simulink model "EV_BMS_Simscape"  (R2026b)
settings: Solver=ode23t  StopTime=5000  MaxStep=1
values from neighbouring files (symbols this model uses):
  thr = struct('pack', Inf, 'curr', Inf, 'innov', Inf, 'noise', Inf)    [simulate_charging_simulink.m]
undefined symbols (not defined in the file or in its folder): ac, bp, defence, seed_atk, seed_meas, seed_u
libraries: nesl_utility x18, evbms_lib x5, fl_lib x1
settings Model: Creator=yugagarwal105  LastModifiedBy=yugagarwal105
settings SimscapeCC: SimscapeLogType=all  SimscapeNominalValues="[{\"value\":\"1\",\"unit\":\"A\"},{\"value\":\"1\",\"unit\":\"bar\"},{\"value\":\"1\",\"unit\":\"cm^2\"},{\"value\":\"1\",\"unit\":\"cm^3/s\"},{\"value\":\"1\",\"unit\":\"kJ/kg\"},{\"value\":\"1\",\"unit\":\"kW\"},{\"value\":\"1\",\"unit\":\"l\"},{\"value\":\"1\",\"unit\":\"N\"},{\"value\":\"1\",\"unit\":\"N*m\"},{\"value\":\"1\",\"unit\":\"V\"},{\"value\":\"0.001\",\"unit\":\"Wb\"}]"  SimscapeUseEnergyAccounting=off

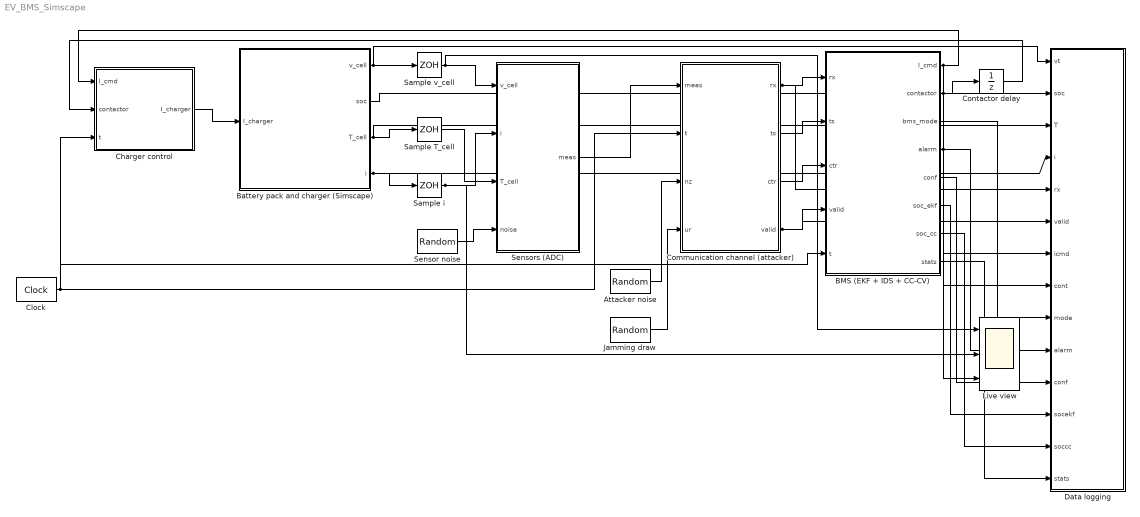
== system EV_BMS_Simscape ==
  Attacker noise : RandomNumber  Mean=zeros(1,4)  Variance=ones(1,4)  Seed=seed_atk  SampleTime=1
  BMS (EKF + IDS + CC-CV) : MATLAB Function  TreatAsAtomicUnit=on
  Battery pack and charger (Simscape) : Subsystem
      mask Display: port_label('input',1,'I charger');port_label('output',1,'V cells');port_label('output',2,'SoC');port_label('output',3,'T cells');port_label('output',4,'I pack');
  Charger control : Subsystem
      mask Display: port_label('input',1,'I cmd');port_label('input',2,'contactor');port_label('input',3,'t');port_label('output',1,'I');
  Clock : DigitalClock
  Communication channel (attacker) : MATLAB Function  TreatAsAtomicUnit=on
  Contactor delay : UnitDelay  InitialCondition=1
  Data logging : Subsystem
      mask Display: disp('Data logging\n(To Workspace)');
  Jamming draw : UniformRandomNumber  Minimum=0  Seed=seed_u  SampleTime=1
  Live view : Scope  NumInputPorts=3
  Sample T_cell : ZeroOrderHold
  Sample i : ZeroOrderHold
  Sample v_cell : ZeroOrderHold
  Sensor noise : RandomNumber  Mean=zeros(1,10)  Variance=ones(1,10)  Seed=seed_meas  SampleTime=1
  Sensors (ADC) : MATLAB Function  TreatAsAtomicUnit=on
  wires:
  Charger control/1(I_charger) -> Battery pack and charger (Simscape)/1(I_charger)
  Battery pack and charger (Simscape)/1(v_cell) -> Sample v_cell/1, Data logging/1(vt)
  Battery pack and charger (Simscape)/4(i) -> Sample i/1, Data logging/4(i)
  Battery pack and charger (Simscape)/3(T_cell) -> Sample T_cell/1, Data logging/3(T)
  Sample v_cell/1 -> Sensors (ADC)/1(v_cell), Live view/1
  Sample i/1 -> Sensors (ADC)/2(i), Live view/2
  Sample T_cell/1 -> Sensors (ADC)/3(T_cell)
  Sensor noise/1 -> Sensors (ADC)/4(noise)
  Sensors (ADC)/1(meas) -> Communication channel (attacker)/1(meas)
  Clock/1 -> Communication channel (attacker)/2(t), BMS (EKF + IDS + CC-CV)/5(t), Charger control/3(t)
  Attacker noise/1 -> Communication channel (attacker)/3(nz)
  Jamming draw/1 -> Communication channel (attacker)/4(ur)
  Communication channel (attacker)/1(rx) -> BMS (EKF + IDS + CC-CV)/1(rx), Data logging/5(rx)
  Communication channel (attacker)/2(ts) -> BMS (EKF + IDS + CC-CV)/2(ts)
  Communication channel (attacker)/3(ctr) -> BMS (EKF + IDS + CC-CV)/3(ctr)
  Communication channel (attacker)/4(valid) -> BMS (EKF + IDS + CC-CV)/4(valid), Data logging/6(valid)
  BMS (EKF + IDS + CC-CV)/1(I_cmd) -> Charger control/1(I_cmd), Data logging/7(icmd)
  BMS (EKF + IDS + CC-CV)/2(contactor) -> Contactor delay/1, Data logging/8(cont)
  Contactor delay/1 -> Charger control/2(contactor)
  Battery pack and charger (Simscape)/2(soc) -> Data logging/2(soc)
  BMS (EKF + IDS + CC-CV)/3(bms_mode) -> Data logging/9(mode)
  BMS (EKF + IDS + CC-CV)/4(alarm) -> Data logging/10(alarm), Live view/3
  BMS (EKF + IDS + CC-CV)/5(conf) -> Data logging/11(conf)
  BMS (EKF + IDS + CC-CV)/6(soc_ekf) -> Data logging/12(socekf)
  BMS (EKF + IDS + CC-CV)/7(soc_cc) -> Data logging/13(soccc)
  BMS (EKF + IDS + CC-CV)/8(stats) -> Data logging/14(stats)

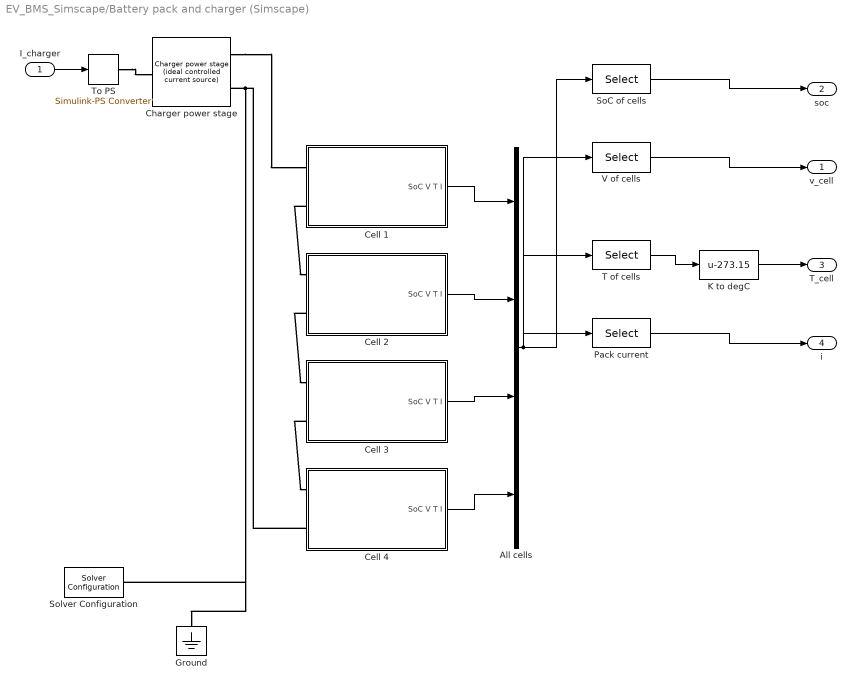
== system EV_BMS_Simscape/Battery pack and charger (Simscape) ==
  I_charger : Inport
  All cells : Mux
  Cell 1 : Subsystem
      mask Display: disp('Li-ion cell 1\nSoC0 = 0.20');port_label('LConn',1,'+');port_label('LConn',2,'-');
  Cell 2 : Subsystem
      mask Display: disp('Li-ion cell 2\nSoC0 = 0.24');port_label('LConn',1,'+');port_label('LConn',2,'-');
  Cell 3 : Subsystem
      mask Display: disp('Li-ion cell 3\nSoC0 = 0.21');port_label('LConn',1,'+');port_label('LConn',2,'-');
  Cell 4 : Subsystem
      mask Display: disp('Li-ion cell 4\nSoC0 = 0.20');port_label('LConn',1,'+');port_label('LConn',2,'-');
  Charger power stage : evbms_lib/Charger power stage (ideal controlled current source)  i_specify=off  i_priority=None  i=0 A  i_nominal_specify=off  i_nominal_value=1  i_nominal_unit=A  v_specify=off  v_priority=None  v=0 V  v_nominal_specify=off  v_nominal_value=1  v_nominal_unit=V
  Ground : fl_lib/Electrical/Electrical Elements/Electrical Reference
  K to degC : Bias  Bias=-273.15  SaturateOnIntegerOverflow=off
  Pack current : Selector  InputPortWidth=16  IndexOptions=Index vector (dialog)  Indices=[4]  OutputSizes=1
  SoC of cells : Selector  InputPortWidth=16  IndexOptions=Index vector (dialog)  Indices=[1 5 9 13]  OutputSizes=1
  Solver Configuration : nesl_utility/Solver Configuration  PhysicalDomain=network_engine_domain  SubClassName=solver  LeftPortType=input  RightPortType=generic  Tones=[]  Harmonics=[]  SimulateNoise=off  Profile=off  UseLocalSampling=off  EnableSwitchedLinearOptims=on  FrequencyDomain=off  UseCCode=off  RelTol=0.001  AbsTol=0.001  MinStep=1e-09  ToWorkspace=off  RevertToSquareIcSolve=off  NumHomotopyIterations=100  PhasorMode=off  PhasorModeNumHarmonics=1  ConsistencySolver=NEWTON_XTOL_AFTER_FTOL  CanonicalOrdering=CANONICAL  OptimizeIntermediates=OPTIMIZED  MulticoreSolverChoice=BACKWARD_EULER  IndexReductionMethod=DerivativeReplacement  DoDC=off  ResidualTolerance=1e-09  ConsistencyTolSource=GLOBAL  ConsistencyAbsTol=0.001  ConsistencyRelTol=0.001  ConsistencyTolFactor=0.001  UseLocalSolver=off  LocalSolverChoice=NE_BACKWARD_EULER_ADVANCER  ResolveIndetEquations=on  FunctionEvalNumThread=1  LocalSolverSampleTime=0.001  DoFixedCost=off  MaxNonlinIter=3  MaxModeIter=2  ComputeImpulses=off  ImpulseIterations=2  LinearAlgebra=auto  LinearAlgebraNumThread=0  EquationFormulation=NE_TIME_EF  DelaysMemoryBudget=1024  AutomaticFiltering=on  FilteringTimeConstant=0.001  PartitionStorageMethod=AS_NEEDED  PartitionMemoryBudget=1024  PartitionMethod=BALANCED  MultibodyUseLocalSolver=off  MultibodyLocalSolverChoice=ODE1  MultibodyLocalSolverSampleTime=0.001
  T of cells : Selector  InputPortWidth=16  IndexOptions=Index vector (dialog)  Indices=[3 7 11 15]  OutputSizes=1
  To PS : nesl_utility/Simulink-PS Converter  PhysicalDomain=network_engine_domain  SubClassName=ps_input  LeftPortType=input  RightPortType=output  PseudoPeriodic=off  Frequencies=[]  NoiseDistribution=none  NoiseParameters=[]  Unit=A  AffineConversion=off  FilteringAndDerivatives=provide  SimscapeFilterOrder=1  InputFilterTimeConstant=0.001  UdotUserProvided=0
  V of cells : Selector  InputPortWidth=16  IndexOptions=Index vector (dialog)  Indices=[2 6 10 14]  OutputSizes=1
  v_cell : Outport
  soc : Outport  Port=2
  T_cell : Outport  Port=3
  i : Outport  Port=4
  wires:
  I_charger/1 -> To PS/1
  Cell 1/1(SoC V T I) -> All cells/1
  Cell 2/1(SoC V T I) -> All cells/2
  Cell 3/1(SoC V T I) -> All cells/3
  Cell 4/1(SoC V T I) -> All cells/4
  All cells/1 -> SoC of cells/1, V of cells/1, T of cells/1, Pack current/1
  SoC of cells/1 -> soc/1
  V of cells/1 -> v_cell/1
  T of cells/1 -> K to degC/1
  K to degC/1 -> T_cell/1
  Pack current/1 -> i/1
  connections:
  To PS/RConn1 -- Charger power stage/LConn1
  Charger power stage/RConn1 -- Cell 1/LConn1
  Cell 1/LConn2 -- Cell 2/LConn1
  Cell 2/LConn2 -- Cell 3/LConn1
  Cell 3/LConn2 -- Cell 4/LConn1
  Cell 4/LConn2 -- Ground/LConn1 -- Charger power stage/RConn2 -- Solver Configuration/RConn1

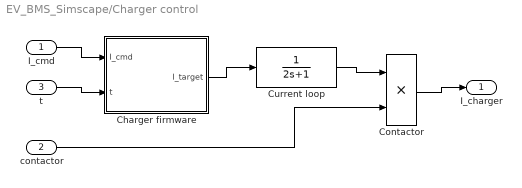
== system EV_BMS_Simscape/Charger control ==
  I_cmd : Inport
  contactor : Inport  Port=2
  t : Inport  Port=3
  Charger firmware : MATLAB Function  TreatAsAtomicUnit=on
  Contactor : Product
  Current loop : TransferFcn  Numerator=1  Denominator=[2 1]
  I_charger : Outport
  wires:
  I_cmd/1 -> Charger firmware/1(I_cmd)
  t/1 -> Charger firmware/2(t)
  Charger firmware/1(I_target) -> Current loop/1
  Current loop/1 -> Contactor/1
  contactor/1 -> Contactor/2
  Contactor/1 -> I_charger/1

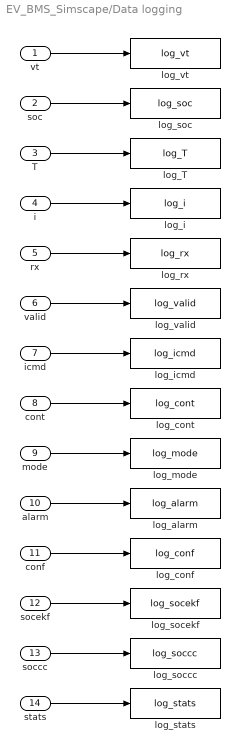
== system EV_BMS_Simscape/Data logging ==
  vt : Inport
  soc : Inport  Port=2
  T : Inport  Port=3
  i : Inport  Port=4
  rx : Inport  Port=5
  valid : Inport  Port=6
  icmd : Inport  Port=7
  cont : Inport  Port=8
  mode : Inport  Port=9
  alarm : Inport  Port=10
  conf : Inport  Port=11
  socekf : Inport  Port=12
  soccc : Inport  Port=13
  stats : Inport  Port=14
  log_T : ToWorkspace  VariableName=log_T  SampleTime=1
      settings: Save2DSignal=2-D array (concatenate along first dimension)
  log_alarm : ToWorkspace  VariableName=log_alarm  SampleTime=1
      settings: Save2DSignal=2-D array (concatenate along first dimension)
  log_conf : ToWorkspace  VariableName=log_conf  SampleTime=1
      settings: Save2DSignal=2-D array (concatenate along first dimension)
  log_cont : ToWorkspace  VariableName=log_cont  SampleTime=1
      settings: Save2DSignal=2-D array (concatenate along first dimension)
  log_i : ToWorkspace  VariableName=log_i  SampleTime=1
      settings: Save2DSignal=2-D array (concatenate along first dimension)
  log_icmd : ToWorkspace  VariableName=log_icmd  SampleTime=1
      settings: Save2DSignal=2-D array (concatenate along first dimension)
  log_mode : ToWorkspace  VariableName=log_mode  SampleTime=1
      settings: Save2DSignal=2-D array (concatenate along first dimension)
  log_rx : ToWorkspace  VariableName=log_rx  SampleTime=1
      settings: Save2DSignal=2-D array (concatenate along first dimension)
  log_soc : ToWorkspace  VariableName=log_soc  SampleTime=1
      settings: Save2DSignal=2-D array (concatenate along first dimension)
  log_soccc : ToWorkspace  VariableName=log_soccc  SampleTime=1
      settings: Save2DSignal=2-D array (concatenate along first dimension)
  log_socekf : ToWorkspace  VariableName=log_socekf  SampleTime=1
      settings: Save2DSignal=2-D array (concatenate along first dimension)
  log_stats : ToWorkspace  VariableName=log_stats  SampleTime=1
      settings: Save2DSignal=2-D array (concatenate along first dimension)
  log_valid : ToWorkspace  VariableName=log_valid  SampleTime=1
      settings: Save2DSignal=2-D array (concatenate along first dimension)
  log_vt : ToWorkspace  VariableName=log_vt  SampleTime=1
      settings: Save2DSignal=2-D array (concatenate along first dimension)
  wires:
  vt/1 -> log_vt/1
  soc/1 -> log_soc/1
  T/1 -> log_T/1
  i/1 -> log_i/1
  rx/1 -> log_rx/1
  valid/1 -> log_valid/1
  icmd/1 -> log_icmd/1
  cont/1 -> log_cont/1
  mode/1 -> log_mode/1
  alarm/1 -> log_alarm/1
  conf/1 -> log_conf/1
  socekf/1 -> log_socekf/1
  soccc/1 -> log_soccc/1
  stats/1 -> log_stats/1

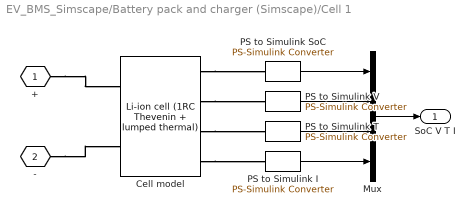
== system EV_BMS_Simscape/Battery pack and charger (Simscape)/Cell 1 ==
  Cell model : evbms_lib/Li-ion cell (1RC Thevenin + lumped thermal)  Q=2.6 A*hr  R0=0.03 Ohm  R1=0.015 Ohm  C1=2000 F  soc0=0.2  soc_bp=[-.1, 0, .05, .1, .2, .3, .4, .5, .6, .7, .8, .9, .95, 1, 1.5]  ocv_tab=[2.8, 3, 3.35, 3.45, 3.55, 3.62, 3.68, 3.74, 3.82, 3.9, 3.98, 4.07, 4.12, 4.2, 5.2] V  Cth=40 J/K  hA=0.05 W/K  Tamb=298.15 K  k_oc=5 W/A  i_specify=off  i_priority=None  i=0 A  i_nominal_specify=off  i_nominal_value=1  i_nominal_unit=A  v_specify=off  v_priority=None  v=0 V  v_nominal_specify=off  v_nominal_value=1  v_nominal_unit=V  v1_specify=off  v1_priority=High  v1=0 V  v1_nominal_specify=off  v1_nominal_value=1  v1_nominal_unit=V  dz_specify=off  dz_priority=High  dz=0  dz_nominal_specify=off  dz_nominal_value=1  dz_nominal_unit=1  dT_specify=off  dT_priority=High  dT=0 K  dT_nominal_specify=off  dT_nominal_value=1  dT_nominal_unit=K
  Mux : Mux
  PS to Simulink I : nesl_utility/PS-Simulink Converter  PhysicalDomain=network_engine_domain  SubClassName=ps_output  LeftPortType=input  RightPortType=output  PseudoPeriodic=off  Frequencies=[]  VectorFormat=inherit  Unit=A  AffineConversion=off
  PS to Simulink SoC : nesl_utility/PS-Simulink Converter  PhysicalDomain=network_engine_domain  SubClassName=ps_output  LeftPortType=input  RightPortType=output  PseudoPeriodic=off  Frequencies=[]  VectorFormat=inherit  Unit=1  AffineConversion=off
  PS to Simulink T : nesl_utility/PS-Simulink Converter  PhysicalDomain=network_engine_domain  SubClassName=ps_output  LeftPortType=input  RightPortType=output  PseudoPeriodic=off  Frequencies=[]  VectorFormat=inherit  Unit=K  AffineConversion=off
  PS to Simulink V : nesl_utility/PS-Simulink Converter  PhysicalDomain=network_engine_domain  SubClassName=ps_output  LeftPortType=input  RightPortType=output  PseudoPeriodic=off  Frequencies=[]  VectorFormat=inherit  Unit=V  AffineConversion=off
  + : PMIOPort  Side=Left
  - : PMIOPort  Port=2  Side=Left
  SoC V T I : Outport
  wires:
  PS to Simulink SoC/1 -> Mux/1
  PS to Simulink V/1 -> Mux/2
  PS to Simulink T/1 -> Mux/3
  PS to Simulink I/1 -> Mux/4
  Mux/1 -> SoC V T I/1
  connections:
  +/RConn1 -- Cell model/LConn1
  -/RConn1 -- Cell model/LConn2
  Cell model/RConn1 -- PS to Simulink SoC/LConn1
  Cell model/RConn2 -- PS to Simulink V/LConn1
  Cell model/RConn3 -- PS to Simulink T/LConn1
  Cell model/RConn4 -- PS to Simulink I/LConn1

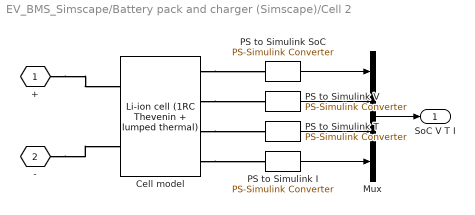
== system EV_BMS_Simscape/Battery pack and charger (Simscape)/Cell 2 ==
  Cell model : evbms_lib/Li-ion cell (1RC Thevenin + lumped thermal)  Q=2.548 A*hr  R0=0.0315 Ohm  R1=0.0156 Ohm  C1=1940 F  soc0=0.24  soc_bp=[-.1, 0, .05, .1, .2, .3, .4, .5, .6, .7, .8, .9, .95, 1, 1.5]  ocv_tab=[2.8, 3, 3.35, 3.45, 3.55, 3.62, 3.68, 3.74, 3.82, 3.9, 3.98, 4.07, 4.12, 4.2, 5.2] V  Cth=40 J/K  hA=0.05 W/K  Tamb=298.15 K  k_oc=5 W/A  i_specify=off  i_priority=None  i=0 A  i_nominal_specify=off  i_nominal_value=1  i_nominal_unit=A  v_specify=off  v_priority=None  v=0 V  v_nominal_specify=off  v_nominal_value=1  v_nominal_unit=V  v1_specify=off  v1_priority=High  v1=0 V  v1_nominal_specify=off  v1_nominal_value=1  v1_nominal_unit=V  dz_specify=off  dz_priority=High  dz=0  dz_nominal_specify=off  dz_nominal_value=1  dz_nominal_unit=1  dT_specify=off  dT_priority=High  dT=0 K  dT_nominal_specify=off  dT_nominal_value=1  dT_nominal_unit=K
  Mux : Mux
  PS to Simulink I : nesl_utility/PS-Simulink Converter  PhysicalDomain=network_engine_domain  SubClassName=ps_output  LeftPortType=input  RightPortType=output  PseudoPeriodic=off  Frequencies=[]  VectorFormat=inherit  Unit=A  AffineConversion=off
  PS to Simulink SoC : nesl_utility/PS-Simulink Converter  PhysicalDomain=network_engine_domain  SubClassName=ps_output  LeftPortType=input  RightPortType=output  PseudoPeriodic=off  Frequencies=[]  VectorFormat=inherit  Unit=1  AffineConversion=off
  PS to Simulink T : nesl_utility/PS-Simulink Converter  PhysicalDomain=network_engine_domain  SubClassName=ps_output  LeftPortType=input  RightPortType=output  PseudoPeriodic=off  Frequencies=[]  VectorFormat=inherit  Unit=K  AffineConversion=off
  PS to Simulink V : nesl_utility/PS-Simulink Converter  PhysicalDomain=network_engine_domain  SubClassName=ps_output  LeftPortType=input  RightPortType=output  PseudoPeriodic=off  Frequencies=[]  VectorFormat=inherit  Unit=V  AffineConversion=off
  + : PMIOPort  Side=Left
  - : PMIOPort  Port=2  Side=Left
  SoC V T I : Outport
  wires:
  PS to Simulink SoC/1 -> Mux/1
  PS to Simulink V/1 -> Mux/2
  PS to Simulink T/1 -> Mux/3
  PS to Simulink I/1 -> Mux/4
  Mux/1 -> SoC V T I/1
  connections:
  +/RConn1 -- Cell model/LConn1
  -/RConn1 -- Cell model/LConn2
  Cell model/RConn1 -- PS to Simulink SoC/LConn1
  Cell model/RConn2 -- PS to Simulink V/LConn1
  Cell model/RConn3 -- PS to Simulink T/LConn1
  Cell model/RConn4 -- PS to Simulink I/LConn1

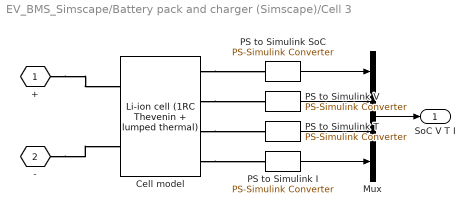
== system EV_BMS_Simscape/Battery pack and charger (Simscape)/Cell 3 ==
  Cell model : evbms_lib/Li-ion cell (1RC Thevenin + lumped thermal)  Q=2.626 A*hr  R0=0.0291 Ohm  R1=0.0147 Ohm  C1=2040 F  soc0=0.21  soc_bp=[-.1, 0, .05, .1, .2, .3, .4, .5, .6, .7, .8, .9, .95, 1, 1.5]  ocv_tab=[2.8, 3, 3.35, 3.45, 3.55, 3.62, 3.68, 3.74, 3.82, 3.9, 3.98, 4.07, 4.12, 4.2, 5.2] V  Cth=40 J/K  hA=0.05 W/K  Tamb=298.15 K  k_oc=5 W/A  i_specify=off  i_priority=None  i=0 A  i_nominal_specify=off  i_nominal_value=1  i_nominal_unit=A  v_specify=off  v_priority=None  v=0 V  v_nominal_specify=off  v_nominal_value=1  v_nominal_unit=V  v1_specify=off  v1_priority=High  v1=0 V  v1_nominal_specify=off  v1_nominal_value=1  v1_nominal_unit=V  dz_specify=off  dz_priority=High  dz=0  dz_nominal_specify=off  dz_nominal_value=1  dz_nominal_unit=1  dT_specify=off  dT_priority=High  dT=0 K  dT_nominal_specify=off  dT_nominal_value=1  dT_nominal_unit=K
  Mux : Mux
  PS to Simulink I : nesl_utility/PS-Simulink Converter  PhysicalDomain=network_engine_domain  SubClassName=ps_output  LeftPortType=input  RightPortType=output  PseudoPeriodic=off  Frequencies=[]  VectorFormat=inherit  Unit=A  AffineConversion=off
  PS to Simulink SoC : nesl_utility/PS-Simulink Converter  PhysicalDomain=network_engine_domain  SubClassName=ps_output  LeftPortType=input  RightPortType=output  PseudoPeriodic=off  Frequencies=[]  VectorFormat=inherit  Unit=1  AffineConversion=off
  PS to Simulink T : nesl_utility/PS-Simulink Converter  PhysicalDomain=network_engine_domain  SubClassName=ps_output  LeftPortType=input  RightPortType=output  PseudoPeriodic=off  Frequencies=[]  VectorFormat=inherit  Unit=K  AffineConversion=off
  PS to Simulink V : nesl_utility/PS-Simulink Converter  PhysicalDomain=network_engine_domain  SubClassName=ps_output  LeftPortType=input  RightPortType=output  PseudoPeriodic=off  Frequencies=[]  VectorFormat=inherit  Unit=V  AffineConversion=off
  + : PMIOPort  Side=Left
  - : PMIOPort  Port=2  Side=Left
  SoC V T I : Outport
  wires:
  PS to Simulink SoC/1 -> Mux/1
  PS to Simulink V/1 -> Mux/2
  PS to Simulink T/1 -> Mux/3
  PS to Simulink I/1 -> Mux/4
  Mux/1 -> SoC V T I/1
  connections:
  +/RConn1 -- Cell model/LConn1
  -/RConn1 -- Cell model/LConn2
  Cell model/RConn1 -- PS to Simulink SoC/LConn1
  Cell model/RConn2 -- PS to Simulink V/LConn1
  Cell model/RConn3 -- PS to Simulink T/LConn1
  Cell model/RConn4 -- PS to Simulink I/LConn1

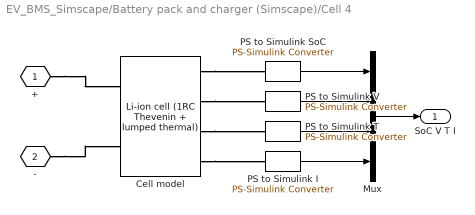
== system EV_BMS_Simscape/Battery pack and charger (Simscape)/Cell 4 ==
  Cell model : evbms_lib/Li-ion cell (1RC Thevenin + lumped thermal)  Q=2.574 A*hr  R0=0.0306 Ohm  R1=0.01515 Ohm  C1=2000 F  soc0=0.2  soc_bp=[-.1, 0, .05, .1, .2, .3, .4, .5, .6, .7, .8, .9, .95, 1, 1.5]  ocv_tab=[2.8, 3, 3.35, 3.45, 3.55, 3.62, 3.68, 3.74, 3.82, 3.9, 3.98, 4.07, 4.12, 4.2, 5.2] V  Cth=40 J/K  hA=0.05 W/K  Tamb=298.15 K  k_oc=5 W/A  i_specify=off  i_priority=None  i=0 A  i_nominal_specify=off  i_nominal_value=1  i_nominal_unit=A  v_specify=off  v_priority=None  v=0 V  v_nominal_specify=off  v_nominal_value=1  v_nominal_unit=V  v1_specify=off  v1_priority=High  v1=0 V  v1_nominal_specify=off  v1_nominal_value=1  v1_nominal_unit=V  dz_specify=off  dz_priority=High  dz=0  dz_nominal_specify=off  dz_nominal_value=1  dz_nominal_unit=1  dT_specify=off  dT_priority=High  dT=0 K  dT_nominal_specify=off  dT_nominal_value=1  dT_nominal_unit=K
  Mux : Mux
  PS to Simulink I : nesl_utility/PS-Simulink Converter  PhysicalDomain=network_engine_domain  SubClassName=ps_output  LeftPortType=input  RightPortType=output  PseudoPeriodic=off  Frequencies=[]  VectorFormat=inherit  Unit=A  AffineConversion=off
  PS to Simulink SoC : nesl_utility/PS-Simulink Converter  PhysicalDomain=network_engine_domain  SubClassName=ps_output  LeftPortType=input  RightPortType=output  PseudoPeriodic=off  Frequencies=[]  VectorFormat=inherit  Unit=1  AffineConversion=off
  PS to Simulink T : nesl_utility/PS-Simulink Converter  PhysicalDomain=network_engine_domain  SubClassName=ps_output  LeftPortType=input  RightPortType=output  PseudoPeriodic=off  Frequencies=[]  VectorFormat=inherit  Unit=K  AffineConversion=off
  PS to Simulink V : nesl_utility/PS-Simulink Converter  PhysicalDomain=network_engine_domain  SubClassName=ps_output  LeftPortType=input  RightPortType=output  PseudoPeriodic=off  Frequencies=[]  VectorFormat=inherit  Unit=V  AffineConversion=off
  + : PMIOPort  Side=Left
  - : PMIOPort  Port=2  Side=Left
  SoC V T I : Outport
  wires:
  PS to Simulink SoC/1 -> Mux/1
  PS to Simulink V/1 -> Mux/2
  PS to Simulink T/1 -> Mux/3
  PS to Simulink I/1 -> Mux/4
  Mux/1 -> SoC V T I/1
  connections:
  +/RConn1 -- Cell model/LConn1
  -/RConn1 -- Cell model/LConn2
  Cell model/RConn1 -- PS to Simulink SoC/LConn1
  Cell model/RConn2 -- PS to Simulink V/LConn1
  Cell model/RConn3 -- PS to Simulink T/LConn1
  Cell model/RConn4 -- PS to Simulink I/LConn1

== matlab function EV_BMS_Simscape/Sensors (ADC) ==
  data: v_cell input; meas output; i input; T_cell input; noise input; bp parameter
function meas = adc(v_cell, i, T_cell, noise, bp)
meas = adc_step(v_cell, i, T_cell, noise, bp);

== matlab function EV_BMS_Simscape/Charger control/Charger firmware ==
  data: I_cmd input; I_target output; t input; ac parameter
function I_target = firmware(I_cmd, t, ac)
I_target = charger_fw(I_cmd, t, ac);

== matlab function EV_BMS_Simscape/Communication channel (attacker) ==
  data: meas input; rx output; t input; nz input; ur input; ts output; ctr output; valid output; ac parameter; bp parameter
function [rx, ts, ctr, valid] = channel(meas, t, nz, ur, ac, bp)
[rx, ts, ctr, valid] = attack_step(meas, t, nz, ur, ac, bp);

== matlab function EV_BMS_Simscape/BMS (EKF + IDS + CC-CV) ==
  data: rx input; I_cmd output; ts input; ctr input; valid input; t input; contactor output; bms_mode output; alarm output; conf output; soc_ekf output; soc_cc output; stats output; bp parameter; thr parameter; defence parameter
function [I_cmd, contactor, bms_mode, alarm, conf, soc_ekf, soc_cc, stats] = bms(rx, ts, ctr, valid, t, bp, thr, defence)
[I_cmd, contactor, bms_mode, alarm, conf, soc_ekf, soc_cc, stats] = bms_step(rx, ts, ctr, valid, t, bp, thr, defence);
